simulink model "part4"  (R2018b)
settings: Solver=VariableStepAuto  StartTime=0.0  StopTime=100  RelTol=1e-3
settings Model: Creator=Engineer  LastModifiedBy=Engineer

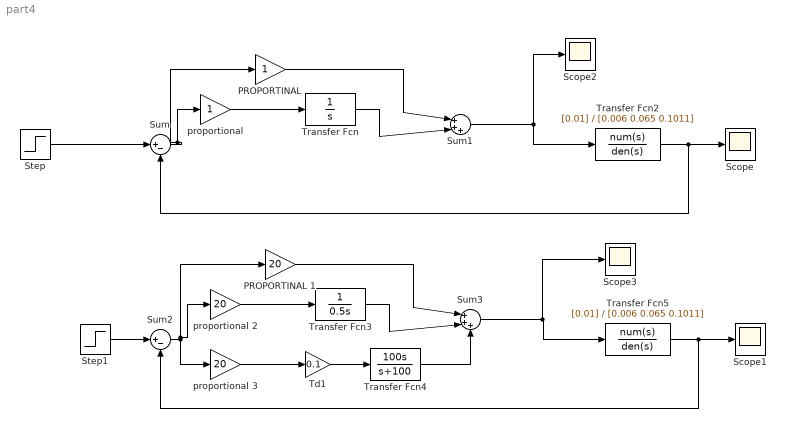
== system part4 ==
  "PROPORTINAL " : Gain
  PROPORTINAL 1 : Gain  Gain=20
  Scope{,1..3} (4 alike) : Scope
  Step : Step  Time=0  SampleTime=0
  Step1 : Step  Time=0  SampleTime=0
  Sum : Sum  Inputs=|+-
  Sum1 : Sum  Inputs=|+++
  Sum2 : Sum  Inputs=|+-
  Sum3 : Sum  Inputs=|+++
  Td1 : Gain  Gain=0.1
  Transfer Fcn : TransferFcn  Denominator=[1 0]
  Transfer Fcn2 : TransferFcn  Numerator=[0.01]  Denominator=[0.006 0.065 0.1011]
  Transfer Fcn3 : TransferFcn  Denominator=[0.5 0]
  Transfer Fcn4 : TransferFcn  Numerator=[100 0]  Denominator=[1 100]
  Transfer Fcn5 : TransferFcn  Numerator=[0.01]  Denominator=[0.006 0.065 0.1011]
  "proportional " : Gain
  proportional 2 : Gain  Gain=20
  proportional 3 : Gain  Gain=20
  wires:
  Sum/1 -> "PROPORTINAL "/1, "proportional "/1
  "proportional "/1 -> Transfer Fcn/1
  Step/1 -> Sum/1
  Sum1/1 -> Transfer Fcn2/1, Scope2/1
  Transfer Fcn2/1 -> Sum/2, Scope/1
  "PROPORTINAL "/1 -> Sum1/1
  Transfer Fcn/1 -> Sum1/2
  Transfer Fcn3/1 -> Sum3/2
  proportional 3/1 -> Td1/1
  PROPORTINAL 1/1 -> Sum3/1
  Transfer Fcn5/1 -> Sum2/2, Scope1/1
  Sum3/1 -> Scope3/1, Transfer Fcn5/1
  Sum2/1 -> PROPORTINAL 1/1, proportional 2/1, proportional 3/1
  Step1/1 -> Sum2/1
  proportional 2/1 -> Transfer Fcn3/1
  Transfer Fcn4/1 -> Sum3/3
  Td1/1 -> Transfer Fcn4/1
